simulink model "part3"  (R2018b)
settings: Solver=VariableStepAuto  StartTime=0.0  StopTime=50  MaxStep=1/60  RelTol=1e-3
settings Model: Creator=Engineer  LastModifiedBy=Engineer

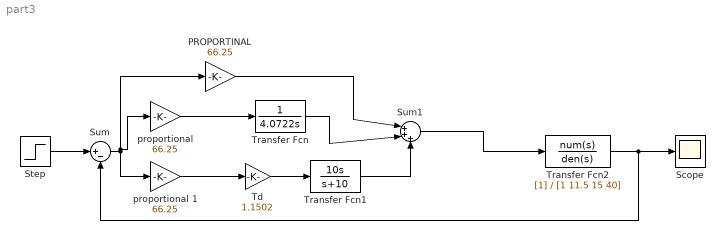
== system part3 ==
  "PROPORTINAL " : Gain  Gain=66.25
  Scope : Scope
  Step : Step  Time=0  SampleTime=0
  Sum : Sum  Inputs=|+-
  Sum1 : Sum  Inputs=|+++
  Td : Gain  Gain=1.1502
  Transfer Fcn : TransferFcn  Denominator=[4.0722 0]
  Transfer Fcn1 : TransferFcn  Numerator=[10 0]  Denominator=[1 10]
  Transfer Fcn2 : TransferFcn  Denominator=[1 11.5 15 40]
  "proportional " : Gain  Gain=66.25
  proportional 1 : Gain  Gain=66.25
  wires:
  proportional 1/1 -> Td/1
  Td/1 -> Transfer Fcn1/1
  Sum/1 -> "PROPORTINAL "/1, "proportional "/1, proportional 1/1
  Step/1 -> Sum/1
  Sum1/1 -> Transfer Fcn2/1
  "proportional "/1 -> Transfer Fcn/1
  Transfer Fcn2/1 -> Sum/2, Scope/1
  Transfer Fcn1/1 -> Sum1/3
  "PROPORTINAL "/1 -> Sum1/1
  Transfer Fcn/1 -> Sum1/2
